simulink model "cartesian_impedance_control"  (R2022b)
settings: Solver=FixedStepDiscrete  StartTime=0.0  StopTime=inf  FixedStep=0.001  RelTol=1e-3
PreLoadFcn:
  | set_param(gcs, 'RTWSystemTargetFile', 'franka_emika_panda.tlc');
  | 
  | demos_common_configs();
  | collision_behavior = ones(1,52)*100;
libraries: franka_simulink_library x5
settings Model: SimulationMode=external  ExtModeTrigDuration=10000  Creator=vasi_ko  LastModifiedBy=rsladmin
settings SolverCC: AlgebraicLoopSolver=TrustRegion
settings DataIOCC: LimitDataPoints=on  SaveFormat=Array  ReturnWorkspaceOutputs=off
settings OptimizationCC: EnhancedBackFolding=on  OptimizeBlockOrder=speed  DifferentSizesBufferReuse=on  OptimizationCustomize=off
settings DebuggingCC: SolverPrmCheckMsg=warning  ParameterTunabilityLossMsg=error  UnconnectedInputMsg=warning  UnconnectedOutputMsg=warning  UnconnectedLineMsg=warning  SFUnexpectedBacktrackingDiag=warning  SFNoUnconditionalDefaultTransitionDiag=warning  SFExecutionAtInitializationDiag=none  SFMachineParentedDataDiag=warning  ArithmeticOperatorsInVariantConditions=warning
settings HardwareCC: ProdBitPerLong=64  ProdHWDeviceType=Intel->x86-64 (Linux 64)
settings ModelReferenceCC: EnableRefExpFcnMdlSchedulingChecks=on  PropagateSignalLabelsOutOfModel=off
settings SFSimCC: SimUseLocalCustomCode=off  MATLABDynamicMemAlloc=off  CustomCodeUndefinedFunction=UseInterfaceOnly  SimTargetLang=C++
settings RTWCC: SystemTargetFile=franka_emika_panda.tlc  RTWUseLocalCustomCode=off  Toolchain=Franka Simulink | gmake (64-bit linux)  BuildConfiguration=Faster Runs  TargetLang=C++
settings CodeAppCC: OperatorAnnotations=on
settings STFCustomTargetCC: TargetLangStandard=C99 (ISO)  ModelReferenceCompliant=off  MatFileLogging=on  GRTInterface=on  UseToolchainInfoCompliant=on  SystemTargetFile=franka_emika_panda.tlc
settings GRTTargetCC: ModelReferenceCompliant=off  ParMdlRefBuildCompliant=off  CompOptLevelCompliant=off  ConcurrentExecutionCompliant=off  CombineOutputUpdateFcns=off  CPPClassGenCompliant=off  GRTInterface=on  ExtModeStaticAlloc=on  ExtModeTransport=1  ExtModeMexFile=ext_xcp  ExtModeIntrfLevel=Level2 - Open
settings ConfigComp: CovMetricSettings=dw  CovSaveCumulativeToWorkspaceVar=on  CovSaveSingleToWorkspaceVar=on  CovExternalEMLEnable=off  CovSFcnEnable=off

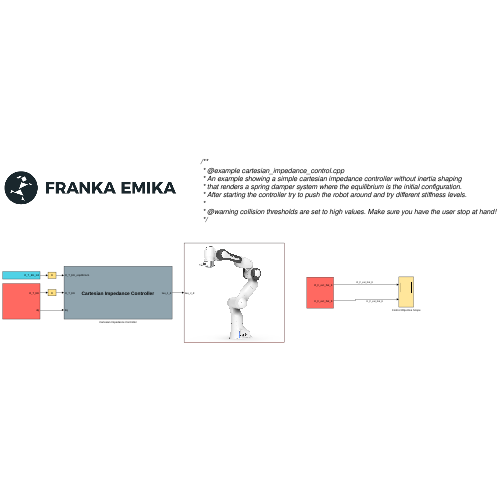
[thumbnail: Simulink's stored preview of the top-level diagram]
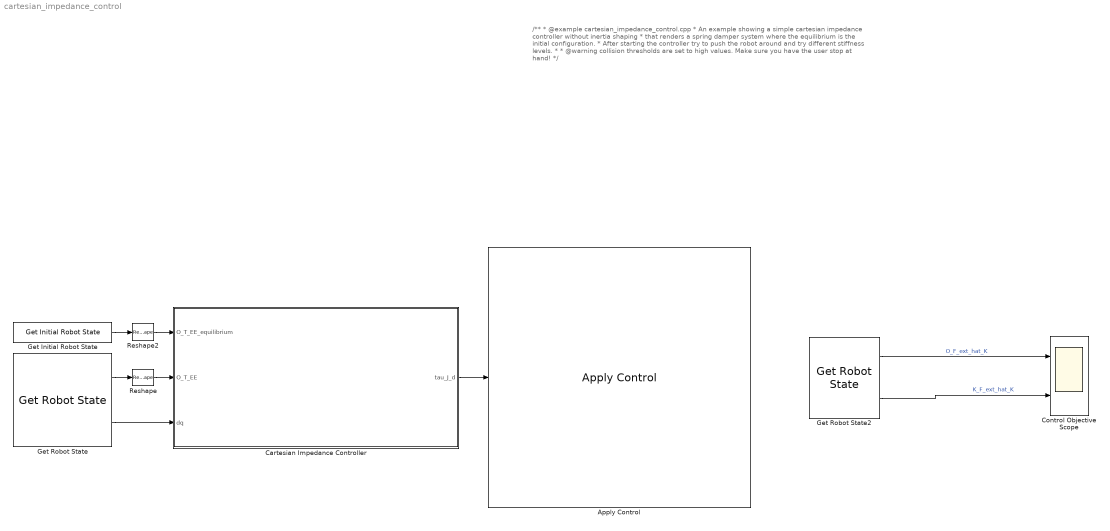
== system cartesian_impedance_control ==
  note: /**
      |  * @example cartesian_impedance_control.cpp
      |  * An example showing a simple cartesian impedance controller without inertia shaping
      |  * that renders a spring damper system where the equilibrium is the initial configuration.
      |  * After starting the controller try to push the robot around and try different stiffness levels.
      |  *
      |  * @warning collision thresholds are set to high values. Make sure you have the user stop at hand!
      |  */
  Apply Control : franka_simulink_library/Apply Control  robot_ip=robot_ip  gripper_attached=off  control_mode=Torque Control  controller_choice=Joint Impedance Controller  elbow_control=on  collision_thresholds=100*ones(1,52)  joint_impedance=joint_impedance  cartesian_impedance=cartesian_impedance  load_inertia=load_inertia  EE_T_K=EE_T_K  init_joint_configuration_req=on  init_joint_configuration=[0, -pi/4, 0, -3 * pi/4, 0, pi/2, pi/4]
      settings: SourceProductName=Franka Emika Simulink Support Package
  Cartesian Impedance Controller : Subsystem
      mask Display:
      | disp('{\bf\fontsize{18}Cartesian Impedance Controller}', 'texmode','on');
      | 
      | block_icon('Controller')
      | 
      | port_label('output',1,'tau_J_d');
      | 
      | port_label('input',1,'O_T_EE_equilibrium');
      | port_label('input',2,'O_T_EE');
      | port_label('input',3,'dq');
  Control Objective Scope : Scope  NumInputPorts=2
  Get Initial Robot State : franka_simulink_library/Get Initial Robot State  robot_ip=robot_ip  signals_requested='O_T_EE'
      settings: SourceProductName=Franka Emika Simulink Support Package
  Get Robot State : franka_simulink_library/Get Robot State  robot_ip=robot_ip  signals_requested='O_T_EE dq'
      settings: SourceProductName=Franka Emika Simulink Support Package
  Get Robot State2 : franka_simulink_library/Get Robot State  robot_ip=robot_ip  signals_requested='O_F_ext_hat_K K_F_ext_hat_K'
      settings: SourceProductName=Franka Emika Simulink Support Package
  Reshape : Reshape  OutputDimensionality=Customize  OutputDimensions=[4,4]
  Reshape2 : Reshape  OutputDimensionality=Customize  OutputDimensions=[4,4]
  wires:
  Cartesian Impedance Controller/1(tau_J_d) -> Apply Control/1
  Get Initial Robot State/1 -> Reshape2/1
  Get Robot State/1 -> Reshape/1
  Get Robot State/2 -> Cartesian Impedance Controller/3(dq)
  Reshape/1 -> Cartesian Impedance Controller/2(O_T_EE)
  Reshape2/1 -> Cartesian Impedance Controller/1(O_T_EE_equilibrium)
  Get Robot State2/1 -> Control Objective Scope/1  "O_F_ext_hat_K"
  Get Robot State2/2 -> Control Objective Scope/2  "K_F_ext_hat_K"

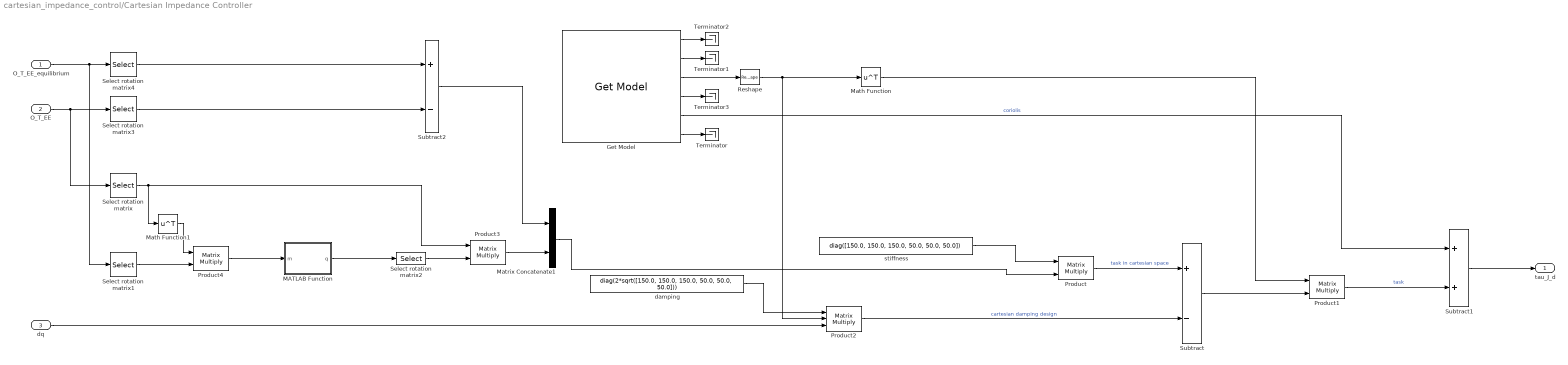
== system cartesian_impedance_control/Cartesian Impedance Controller ==
  O_T_EE_equilibrium : Inport
  O_T_EE : Inport  Port=2
  dq : Inport  Port=3
  Get Model : franka_simulink_library/Get Model  robot_ip=robot_ip
      settings: SourceProductName=Franka Emika Simulink Support Package
  MATLAB Function : MATLAB Function  TreatAsAtomicUnit=on
  Math Function : Math  Operator=transpose  SignedPower=on
  Math Function1 : Math  Operator=transpose  SignedPower=on
  Matrix Concatenate1 : Concatenate
  Product{,1,3..4} (4 alike) : Product  Multiplication=Matrix(*)
  Product2 : Product  Inputs=3  Multiplication=Matrix(*)
  Reshape : Reshape  OutputDimensionality=Customize  OutputDimensions=[6,7]
  Select rotation matrix : Selector  NumberOfDimensions=2  InputPortWidth=3  IndexOptions=Index vector (dialog),Index vector (dialog)  Indices=[1,2,3],[1 2 3]  OutputSizes=1
  Select rotation matrix1 : Selector  NumberOfDimensions=2  InputPortWidth=3  IndexOptions=Index vector (dialog),Index vector (dialog)  Indices=[1,2,3],[1 2 3]  OutputSizes=1
  Select rotation matrix2 : Selector  InputPortWidth=4  IndexOptions=Index vector (dialog)  Indices=[2,3,4]  OutputSizes=1
  Select rotation matrix3 : Selector  NumberOfDimensions=2  InputPortWidth=3  IndexOptions=Index vector (dialog),Index vector (dialog)  Indices=[1,2,3],[4]  OutputSizes=1
  Select rotation matrix4 : Selector  NumberOfDimensions=2  InputPortWidth=3  IndexOptions=Index vector (dialog),Index vector (dialog)  Indices=[1,2,3],[4]  OutputSizes=1
  Subtract : Sum  Inputs=+-
  Subtract1 : Sum
  Subtract2 : Sum  Inputs=+-
  Terminator{,1..3} (4 alike) : Terminator
  damping : Constant  Value=diag(2*sqrt([150.0, 150.0, 150.0, 50.0, 50.0, 50.0]))  VectorParams1D=off
  stiffness : Constant  Value=diag([150.0, 150.0, 150.0, 50.0, 50.0, 50.0])  VectorParams1D=off
  tau_J_d : Outport  VectorParamsAs1DForOutWhenUnconnected=off
  wires:
  Get Model/6 -> Terminator/1
  Get Model/2 -> Terminator1/1
  Get Model/1 -> Terminator2/1
  Get Model/4 -> Terminator3/1
  Get Model/3 -> Reshape/1
  Reshape/1 -> Product2/2, Math Function/1
  stiffness/1 -> Product/1
  Math Function/1 -> Product1/1
  Product/1 -> Subtract/1  "task in cartesian space"
  Product2/1 -> Subtract/2  "cartesian damping design"
  Get Model/5 -> Subtract1/1  "coriolis"
  dq/1 -> Product2/3
  damping/1 -> Product2/1
  Subtract1/1 -> tau_J_d/1
  Product1/1 -> Subtract1/2  "task"
  O_T_EE/1 -> Select rotation matrix3/1, Select rotation matrix/1
  O_T_EE_equilibrium/1 -> Select rotation matrix4/1, Select rotation matrix1/1
  Select rotation matrix4/1 -> Subtract2/1
  Select rotation matrix3/1 -> Subtract2/2
  Subtract2/1 -> Matrix Concatenate1/1
  MATLAB Function/1(q) -> Select rotation matrix2/1
  Product4/1 -> MATLAB Function/1(m)
  Subtract/1 -> Product1/2
  Select rotation matrix2/1 -> Product3/2
  Matrix Concatenate1/1 -> Product/2
  Select rotation matrix/1 -> Math Function1/1, Product3/1
  Product3/1 -> Matrix Concatenate1/2
  Select rotation matrix1/1 -> Product4/2
  Math Function1/1 -> Product4/1

== matlab function cartesian_impedance_control/Cartesian Impedance Controller/MATLAB Function ==
  data: m input; q output
function q = rotm2quat(m)

m00 = m(1,1);
m01 = m(1,2);
m02 = m(1,3);

m10 = m(2,1);
m11 = m(2,2);
m12 = m(2,3);

m20 = m(3,1);
m21 = m(3,2);
m22 = m(3,3);

tr = m00 + m11 + m22;

if (tr > 0) 
  S = sqrt(tr+1.0) * 2; % S=4*qw 
  qw = 0.25 * S;
  qx = (m21 - m12) / S;
  qy = (m02 - m20) / S; 
  qz = (m10 - m01) / S; 
elseif ((m00 > m11) && (m00 > m22))
  S = sqrt(1.0 + m00 - m11 - m22) * 2;  %S=4*qx 
  qw = (m21 - m12) / S;
  qx = 0.25 * S;
  qy = (m01 + m10) / S; 
  qz = (m02 + m20) / S; 
elseif (m11 > m22) 
  S = sqrt(1.0 + m11 - m00 - m22) * 2; % S=4*qy
  qw = (m02 - m20) / S;
  qx = (m01 + m10) / S; 
  qy = 0.25 * S;
  qz = (m12 + m21) / S; 
else 
  S = sqrt(1.0 + m22 - m00 - m11) * 2; % S=4*qz
  qw = (m10 - m01) / S;
  qx = (m02 + m20) / S;
  qy = (m12 + m21) / S;
  qz = 0.25 * S;
end

q = [qw,qx,qy,qz]';
